simulink model "adc083000x2"  (R2016b)
settings: Solver=VariableStepAuto  StartTime=0.0  StopTime=10.0  RelTol=1e-3
libraries: xbsIndex_r4 x22, xps_library x17
settings Model: Creator=qwerty40  LastModifiedBy=qwerty40

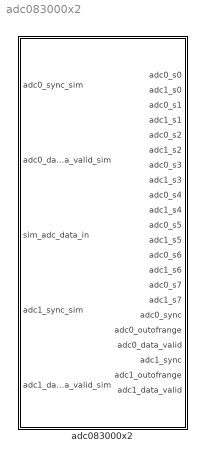
== system adc083000x2 ==
  adc083000x2 : Subsystem  Tag=xps:adc083000x2  mask(adc_083000x2){use_adc0=on, use_adc1=on, demux_adc=off, clock_sync=on, verbose=off, using_ctrl=on, adc_clk_rate=1000, sample_period=1, bit_width=8}
      mask prompts: use_adc0 "Use ZD0K0?"; use_adc1 "Use ZDOK1?"; demux_adc "Demux ADCs by 2?"; clock_sync "Interleave 2 ADC boards?"; verbose "Verbose Block Creation?"; using_ctrl "Add ports for control registers?"; adc_clk_rate "ADC clock rate (MHz)"; sample_period "Sample Period"; bit_width "Output Bit Width"
      mask help:
      | The ADC block converts analog inputs to digital outputs.
      | Every clock cycle, the inputs are sampled and digitized to
      | 8 bit binary point numbers in the range of [-1, 1).
      |
      | Online block-specific documentation: http://casper.berkeley.edu/wiki/Adc083000
      mask init:
      | adc083000_mask;
      mask Help: eval('xlWeb([getenv(''MLIB_ROOT''), ''\doc\html\sys_adc\sys_adc.html''])')

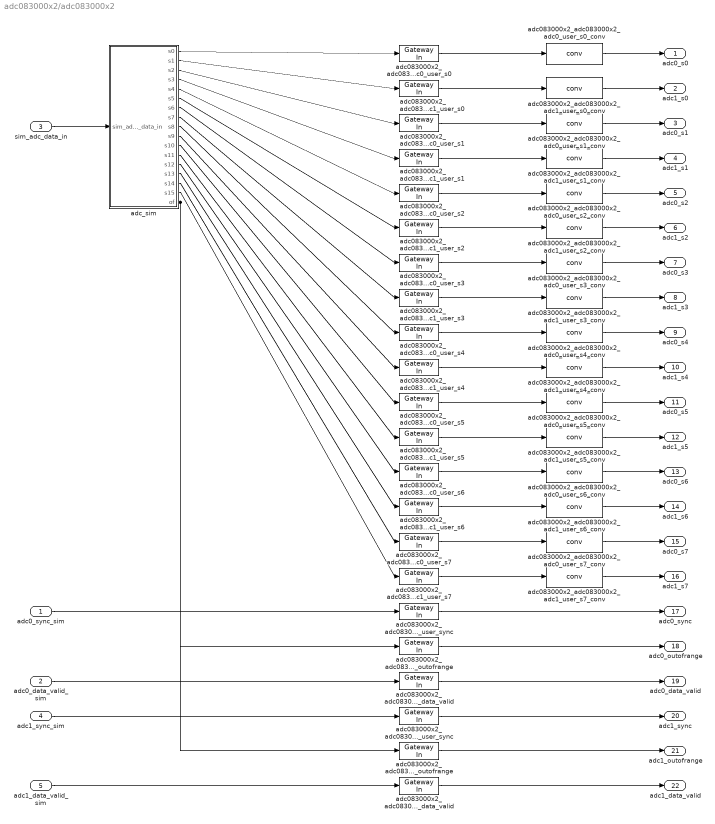
== system adc083000x2/adc083000x2 ==
  adc0_sync_sim : Inport
  adc0_data_valid_sim : Inport  Port=2
  sim_adc_data_in : Inport  Port=3
  adc1_sync_sim : Inport  Port=4
  adc1_data_valid_sim : Inport  Port=5
  adc083000x2_adc083000x2_adc0_user_data_valid : xbsIndex_r4/Gateway In  gui_display_data_type=Fixed-point  arith_type=Unsigned  n_bits=1  bin_pt=0  preci_type=Single  exp_width=8  frac_width=24  rows=1  columns=1  quantization="Round  (unbiased: +/- Inf)"  overflow=Saturate  period=1  UseAsADC=off  ADCChannel='1'  interface=None  automatic_assignment=on  address_offset=hex2dec('00')  intf_name=''  intf_description=''  default_value=0  timing_constraint=None  locs_specified=off  LOCs={}  io_standard={}  inherit_from_input=off  hdl_port=on  dbl_ovrd=off  block_type=gatewayin
  adc083000x2_adc083000x2_adc0_user_outofrange : xbsIndex_r4/Gateway In  gui_display_data_type=Fixed-point  arith_type=Unsigned  n_bits=4  bin_pt=0  preci_type=Single  exp_width=8  frac_width=24  rows=1  columns=1  quantization="Round  (unbiased: +/- Inf)"  overflow=Saturate  period=1  UseAsADC=off  ADCChannel='1'  interface=None  automatic_assignment=on  address_offset=hex2dec('00')  intf_name=''  intf_description=''  default_value=0  timing_constraint=None  locs_specified=off  LOCs={}  io_standard={}  inherit_from_input=off  hdl_port=on  dbl_ovrd=off  block_type=gatewayin
  adc083000x2_adc083000x2_adc0_user_s{0..7} (8 alike) : xbsIndex_r4/Gateway In  gui_display_data_type=Fixed-point  arith_type=Unsigned  n_bits=8  bin_pt=0  preci_type=Single  exp_width=8  frac_width=24  rows=1  columns=1  quantization="Round  (unbiased: +/- Inf)"  overflow=Saturate  period=1  UseAsADC=off  ADCChannel='1'  interface=None  automatic_assignment=on  address_offset=hex2dec('00')  intf_name=''  intf_description=''  default_value=0  timing_constraint=None  locs_specified=off  LOCs={}  io_standard={}  inherit_from_input=off  hdl_port=on  dbl_ovrd=off  block_type=gatewayin
  adc083000x2_adc083000x2_adc0_user_s0_conv : xps_library/ADCs/conv  bit_width=8
  adc083000x2_adc083000x2_adc0_user_s1_conv : xps_library/ADCs/conv  bit_width=8
  adc083000x2_adc083000x2_adc0_user_s2_conv : xps_library/ADCs/conv  bit_width=8
  adc083000x2_adc083000x2_adc0_user_s3_conv : xps_library/ADCs/conv  bit_width=8
  adc083000x2_adc083000x2_adc0_user_s4_conv : xps_library/ADCs/conv  bit_width=8
  adc083000x2_adc083000x2_adc0_user_s5_conv : xps_library/ADCs/conv  bit_width=8
  adc083000x2_adc083000x2_adc0_user_s6_conv : xps_library/ADCs/conv  bit_width=8
  adc083000x2_adc083000x2_adc0_user_s7_conv : xps_library/ADCs/conv  bit_width=8
  adc083000x2_adc083000x2_adc0_user_sync : xbsIndex_r4/Gateway In  gui_display_data_type=Fixed-point  arith_type=Unsigned  n_bits=4  bin_pt=0  preci_type=Single  exp_width=8  frac_width=24  rows=1  columns=1  quantization="Round  (unbiased: +/- Inf)"  overflow=Saturate  period=1  UseAsADC=off  ADCChannel='1'  interface=None  automatic_assignment=on  address_offset=hex2dec('00')  intf_name=''  intf_description=''  default_value=0  timing_constraint=None  locs_specified=off  LOCs={}  io_standard={}  inherit_from_input=off  hdl_port=on  dbl_ovrd=off  block_type=gatewayin
  adc083000x2_adc083000x2_adc1_user_data_valid : xbsIndex_r4/Gateway In  gui_display_data_type=Fixed-point  arith_type=Unsigned  n_bits=1  bin_pt=0  preci_type=Single  exp_width=8  frac_width=24  rows=1  columns=1  quantization="Round  (unbiased: +/- Inf)"  overflow=Saturate  period=1  UseAsADC=off  ADCChannel='1'  interface=None  automatic_assignment=on  address_offset=hex2dec('00')  intf_name=''  intf_description=''  default_value=0  timing_constraint=None  locs_specified=off  LOCs={}  io_standard={}  inherit_from_input=off  hdl_port=on  dbl_ovrd=off  block_type=gatewayin
  adc083000x2_adc083000x2_adc1_user_outofrange : xbsIndex_r4/Gateway In  gui_display_data_type=Fixed-point  arith_type=Unsigned  n_bits=4  bin_pt=0  preci_type=Single  exp_width=8  frac_width=24  rows=1  columns=1  quantization="Round  (unbiased: +/- Inf)"  overflow=Saturate  period=1  UseAsADC=off  ADCChannel='1'  interface=None  automatic_assignment=on  address_offset=hex2dec('00')  intf_name=''  intf_description=''  default_value=0  timing_constraint=None  locs_specified=off  LOCs={}  io_standard={}  inherit_from_input=off  hdl_port=on  dbl_ovrd=off  block_type=gatewayin
  adc083000x2_adc083000x2_adc1_user_s{0..7} (8 alike) : xbsIndex_r4/Gateway In  gui_display_data_type=Fixed-point  arith_type=Unsigned  n_bits=8  bin_pt=0  preci_type=Single  exp_width=8  frac_width=24  rows=1  columns=1  quantization="Round  (unbiased: +/- Inf)"  overflow=Saturate  period=1  UseAsADC=off  ADCChannel='1'  interface=None  automatic_assignment=on  address_offset=hex2dec('00')  intf_name=''  intf_description=''  default_value=0  timing_constraint=None  locs_specified=off  LOCs={}  io_standard={}  inherit_from_input=off  hdl_port=on  dbl_ovrd=off  block_type=gatewayin
  adc083000x2_adc083000x2_adc1_user_s0_conv : xps_library/ADCs/conv  bit_width=8
  adc083000x2_adc083000x2_adc1_user_s1_conv : xps_library/ADCs/conv  bit_width=8
  adc083000x2_adc083000x2_adc1_user_s2_conv : xps_library/ADCs/conv  bit_width=8
  adc083000x2_adc083000x2_adc1_user_s3_conv : xps_library/ADCs/conv  bit_width=8
  adc083000x2_adc083000x2_adc1_user_s4_conv : xps_library/ADCs/conv  bit_width=8
  adc083000x2_adc083000x2_adc1_user_s5_conv : xps_library/ADCs/conv  bit_width=8
  adc083000x2_adc083000x2_adc1_user_s6_conv : xps_library/ADCs/conv  bit_width=8
  adc083000x2_adc083000x2_adc1_user_s7_conv : xps_library/ADCs/conv  bit_width=8
  adc083000x2_adc083000x2_adc1_user_sync : xbsIndex_r4/Gateway In  gui_display_data_type=Fixed-point  arith_type=Unsigned  n_bits=4  bin_pt=0  preci_type=Single  exp_width=8  frac_width=24  rows=1  columns=1  quantization="Round  (unbiased: +/- Inf)"  overflow=Saturate  period=1  UseAsADC=off  ADCChannel='1'  interface=None  automatic_assignment=on  address_offset=hex2dec('00')  intf_name=''  intf_description=''  default_value=0  timing_constraint=None  locs_specified=off  LOCs={}  io_standard={}  inherit_from_input=off  hdl_port=on  dbl_ovrd=off  block_type=gatewayin
  adc_sim : Subsystem  AncestorBlock=xps_library/ADCs/adc_sim  mask(adc_sim){nStreams=16, bit_width=8}
      mask prompts: nStreams "Number of Output Streams"; bit_width "Sample Bit Width"
      mask help:
      | This block simulates the behavior of a demuxed ADC, which takes
      | as input a waveform and returns digital samples in parallel at
      | a slower rate.
      |
      | This block is used to simulate the behavior
      mask init:
      | adc_sim_init(gcb, ...
      |     'nStreams', nStreams, ...
      |     'bit_width', bit_width);
  adc0_s0 : Outport
  adc1_s0 : Outport  Port=2
  adc0_s1 : Outport  Port=3
  adc1_s1 : Outport  Port=4
  adc0_s2 : Outport  Port=5
  adc1_s2 : Outport  Port=6
  adc0_s3 : Outport  Port=7
  adc1_s3 : Outport  Port=8
  adc0_s4 : Outport  Port=9
  adc1_s4 : Outport  Port=10
  adc0_s5 : Outport  Port=11
  adc1_s5 : Outport  Port=12
  adc0_s6 : Outport  Port=13
  adc1_s6 : Outport  Port=14
  adc0_s7 : Outport  Port=15
  adc1_s7 : Outport  Port=16
  adc0_sync : Outport  Port=17
  adc0_outofrange : Outport  Port=18
  adc0_data_valid : Outport  Port=19
  adc1_sync : Outport  Port=20
  adc1_outofrange : Outport  Port=21
  adc1_data_valid : Outport  Port=22
  wires:
  sim_adc_data_in/1 -> adc_sim/1(sim_adc_data_in)
  adc_sim/1(s0) -> adc083000x2_adc083000x2_adc0_user_s0/1
  adc083000x2_adc083000x2_adc0_user_s0/1 -> adc083000x2_adc083000x2_adc0_user_s0_conv/1
  adc083000x2_adc083000x2_adc0_user_s0_conv/1 -> adc0_s0/1
  adc_sim/2(s1) -> adc083000x2_adc083000x2_adc1_user_s0/1
  adc083000x2_adc083000x2_adc1_user_s0/1 -> adc083000x2_adc083000x2_adc1_user_s0_conv/1
  adc083000x2_adc083000x2_adc1_user_s0_conv/1 -> adc1_s0/1
  adc_sim/3(s2) -> adc083000x2_adc083000x2_adc0_user_s1/1
  adc083000x2_adc083000x2_adc0_user_s1/1 -> adc083000x2_adc083000x2_adc0_user_s1_conv/1
  adc083000x2_adc083000x2_adc0_user_s1_conv/1 -> adc0_s1/1
  adc_sim/4(s3) -> adc083000x2_adc083000x2_adc1_user_s1/1
  adc083000x2_adc083000x2_adc1_user_s1/1 -> adc083000x2_adc083000x2_adc1_user_s1_conv/1
  adc083000x2_adc083000x2_adc1_user_s1_conv/1 -> adc1_s1/1
  adc_sim/5(s4) -> adc083000x2_adc083000x2_adc0_user_s2/1
  adc083000x2_adc083000x2_adc0_user_s2/1 -> adc083000x2_adc083000x2_adc0_user_s2_conv/1
  adc083000x2_adc083000x2_adc0_user_s2_conv/1 -> adc0_s2/1
  adc_sim/6(s5) -> adc083000x2_adc083000x2_adc1_user_s2/1
  adc083000x2_adc083000x2_adc1_user_s2/1 -> adc083000x2_adc083000x2_adc1_user_s2_conv/1
  adc083000x2_adc083000x2_adc1_user_s2_conv/1 -> adc1_s2/1
  adc_sim/7(s6) -> adc083000x2_adc083000x2_adc0_user_s3/1
  adc083000x2_adc083000x2_adc0_user_s3/1 -> adc083000x2_adc083000x2_adc0_user_s3_conv/1
  adc083000x2_adc083000x2_adc0_user_s3_conv/1 -> adc0_s3/1
  adc_sim/8(s7) -> adc083000x2_adc083000x2_adc1_user_s3/1
  adc083000x2_adc083000x2_adc1_user_s3/1 -> adc083000x2_adc083000x2_adc1_user_s3_conv/1
  adc083000x2_adc083000x2_adc1_user_s3_conv/1 -> adc1_s3/1
  adc_sim/9(s8) -> adc083000x2_adc083000x2_adc0_user_s4/1
  adc083000x2_adc083000x2_adc0_user_s4/1 -> adc083000x2_adc083000x2_adc0_user_s4_conv/1
  adc083000x2_adc083000x2_adc0_user_s4_conv/1 -> adc0_s4/1
  adc_sim/10(s9) -> adc083000x2_adc083000x2_adc1_user_s4/1
  adc083000x2_adc083000x2_adc1_user_s4/1 -> adc083000x2_adc083000x2_adc1_user_s4_conv/1
  adc083000x2_adc083000x2_adc1_user_s4_conv/1 -> adc1_s4/1
  adc_sim/11(s10) -> adc083000x2_adc083000x2_adc0_user_s5/1
  adc083000x2_adc083000x2_adc0_user_s5/1 -> adc083000x2_adc083000x2_adc0_user_s5_conv/1
  adc083000x2_adc083000x2_adc0_user_s5_conv/1 -> adc0_s5/1
  adc_sim/12(s11) -> adc083000x2_adc083000x2_adc1_user_s5/1
  adc083000x2_adc083000x2_adc1_user_s5/1 -> adc083000x2_adc083000x2_adc1_user_s5_conv/1
  adc083000x2_adc083000x2_adc1_user_s5_conv/1 -> adc1_s5/1
  adc_sim/13(s12) -> adc083000x2_adc083000x2_adc0_user_s6/1
  adc083000x2_adc083000x2_adc0_user_s6/1 -> adc083000x2_adc083000x2_adc0_user_s6_conv/1
  adc083000x2_adc083000x2_adc0_user_s6_conv/1 -> adc0_s6/1
  adc_sim/14(s13) -> adc083000x2_adc083000x2_adc1_user_s6/1
  adc083000x2_adc083000x2_adc1_user_s6/1 -> adc083000x2_adc083000x2_adc1_user_s6_conv/1
  adc083000x2_adc083000x2_adc1_user_s6_conv/1 -> adc1_s6/1
  adc_sim/15(s14) -> adc083000x2_adc083000x2_adc0_user_s7/1
  adc083000x2_adc083000x2_adc0_user_s7/1 -> adc083000x2_adc083000x2_adc0_user_s7_conv/1
  adc083000x2_adc083000x2_adc0_user_s7_conv/1 -> adc0_s7/1
  adc_sim/16(s15) -> adc083000x2_adc083000x2_adc1_user_s7/1
  adc083000x2_adc083000x2_adc1_user_s7/1 -> adc083000x2_adc083000x2_adc1_user_s7_conv/1
  adc083000x2_adc083000x2_adc1_user_s7_conv/1 -> adc1_s7/1
  adc0_sync_sim/1 -> adc083000x2_adc083000x2_adc0_user_sync/1
  adc083000x2_adc083000x2_adc0_user_sync/1 -> adc0_sync/1
  adc_sim/17(of) -> adc083000x2_adc083000x2_adc0_user_outofrange/1, adc083000x2_adc083000x2_adc1_user_outofrange/1
  adc083000x2_adc083000x2_adc0_user_outofrange/1 -> adc0_outofrange/1
  adc0_data_valid_sim/1 -> adc083000x2_adc083000x2_adc0_user_data_valid/1
  adc083000x2_adc083000x2_adc0_user_data_valid/1 -> adc0_data_valid/1
  adc1_sync_sim/1 -> adc083000x2_adc083000x2_adc1_user_sync/1
  adc083000x2_adc083000x2_adc1_user_sync/1 -> adc1_sync/1
  adc083000x2_adc083000x2_adc1_user_outofrange/1 -> adc1_outofrange/1
  adc1_data_valid_sim/1 -> adc083000x2_adc083000x2_adc1_user_data_valid/1
  adc083000x2_adc083000x2_adc1_user_data_valid/1 -> adc1_data_valid/1

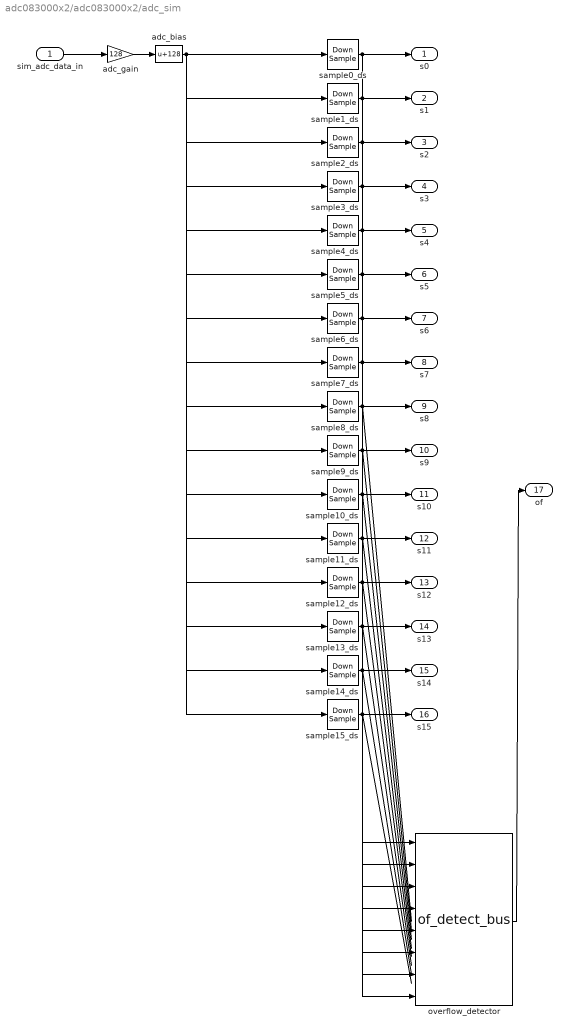
== system adc083000x2/adc083000x2/adc_sim ==
  sim_adc_data_in : Inport
  adc_bias : Bias  Bias=128  SaturateOnIntegerOverflow=on
  adc_gain : Gain  Gain=128
  overflow_detector : xps_library/ADCs/of_detect_bus  nStreams=16  bit_width=8
  sample0_ds : DownSample  N=16  phase=1  smode=Force single rate
  sample10_ds : DownSample  N=16  phase=11  smode=Force single rate
  sample11_ds : DownSample  N=16  phase=12  smode=Force single rate
  sample12_ds : DownSample  N=16  phase=13  smode=Force single rate
  sample13_ds : DownSample  N=16  phase=14  smode=Force single rate
  sample14_ds : DownSample  N=16  phase=15  smode=Force single rate
  sample15_ds : DownSample  N=16  smode=Force single rate
  sample1_ds : DownSample  N=16  phase=2  smode=Force single rate
  sample2_ds : DownSample  N=16  phase=3  smode=Force single rate
  sample3_ds : DownSample  N=16  phase=4  smode=Force single rate
  sample4_ds : DownSample  N=16  phase=5  smode=Force single rate
  sample5_ds : DownSample  N=16  phase=6  smode=Force single rate
  sample6_ds : DownSample  N=16  phase=7  smode=Force single rate
  sample7_ds : DownSample  N=16  phase=8  smode=Force single rate
  sample8_ds : DownSample  N=16  phase=9  smode=Force single rate
  sample9_ds : DownSample  N=16  phase=10  smode=Force single rate
  s0 : Outport
  s1 : Outport  Port=2
  s2 : Outport  Port=3
  s3 : Outport  Port=4
  s4 : Outport  Port=5
  s5 : Outport  Port=6
  s6 : Outport  Port=7
  s7 : Outport  Port=8
  s8 : Outport  Port=9
  s9 : Outport  Port=10
  s10 : Outport  Port=11
  s11 : Outport  Port=12
  s12 : Outport  Port=13
  s13 : Outport  Port=14
  s14 : Outport  Port=15
  s15 : Outport  Port=16
  of : Outport  Port=17
  wires:
  sample15_ds/1 -> s15/1
  sample14_ds/1 -> s14/1
  sample13_ds/1 -> s13/1
  sample12_ds/1 -> s12/1
  sample11_ds/1 -> s11/1
  sample10_ds/1 -> s10/1
  sample9_ds/1 -> s9/1
  sample8_ds/1 -> s8/1
  sample7_ds/1 -> s7/1, overflow_detector/8
  sample6_ds/1 -> s6/1, overflow_detector/7
  sample5_ds/1 -> s5/1, overflow_detector/6
  sample4_ds/1 -> s4/1, overflow_detector/5
  sample3_ds/1 -> s3/1, overflow_detector/4
  sample2_ds/1 -> s2/1, overflow_detector/3
  sample1_ds/1 -> s1/1, overflow_detector/2
  sample0_ds/1 -> s0/1, overflow_detector/1
  adc_bias/1 -> sample15_ds/1, sample14_ds/1, sample13_ds/1, sample12_ds/1, sample11_ds/1, sample10_ds/1, sample9_ds/1, sample8_ds/1, sample7_ds/1, sample6_ds/1, sample5_ds/1, sample4_ds/1, sample3_ds/1, sample2_ds/1, sample1_ds/1, sample0_ds/1
  overflow_detector/1 -> of/1
  adc_gain/1 -> adc_bias/1
  sim_adc_data_in/1 -> adc_gain/1
